simulink model "example_frictions"  (R2023b)
settings: Solver=FixedStepAuto  StartTime=0.0  StopTime=10.0  FixedStep=1/100  RelTol=1e-3
settings Model: Creator=Moi  LastModifiedBy=T0144666
settings OptimizationCC: ReuseModelBlockBuffer=off

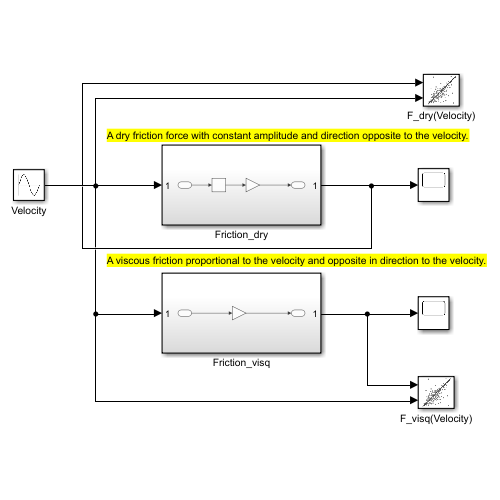
[thumbnail: Simulink's stored preview of the top-level diagram]
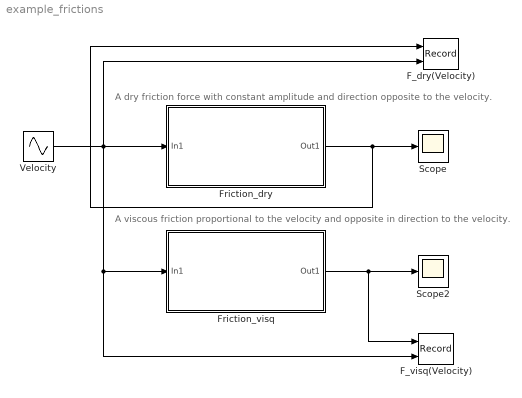
== system example_frictions ==
  note: A dry friction force with constant amplitude and direction opposite to the velocity.
  note: A viscous friction proportional to the velocity and opposite in direction to the velocity.
  F_dry(Velocity) : Record  FileSettingsInternal="{\"entries\":[{\"content\":{\"excelSettings\":{\"content\":{},\"type\":\"Streamout.ExcelSettings\"}},\"type\":\"Streamout.FileSettingStorage\",\"uuid\":\"\"}],\"packageUris\":[\"http:\\/\\/schema.mathworks.com\\/mf0\\/streamout_blocks\\/R2020a\"],\"version\":\"1.0\"}"  Layout=[1 1]  SignalsInternal="{\"entries\":[{\"content\":{\"signals\":[{\"content\":{\"blockPath\":[],\"dimensions\":[1],\"domain\":\"\",\"lineColor\":\"#a2142f\",\"plots\":[1],\"port\":1,\"signalID\":16,\"signalName\":\"frottement_sec\"},\"type\":\"RecordBlkView.Signal\",\"uuid\":\"\"},{\"content\":{\"blockPath\":[],\"dimensions\":[1],\"domain\":\"\",\"lineColor\":\"#139fff\",\"plots\":[1],\"port\":2,\"signalID\":19,\"signalName\":\"vitesse\"},\"type\":\"RecordBlkView.Signal\",\"uuid\":\"\"}]},\"type\":\"RecordBlkView.InputSignals\",\"uuid\":\"\"}],\"packageUris\":[\"http:\\/\\/schema.mathworks.com\\/mf0\\/streamout_blocks\\/R2020a\"],\"version\":\"1.0\"}"  VisualizationBindings="{\"xyplotplugin\":{\"info\":[{\"series\":[{\"bindingParametersList\":[{\"parameter\":\"X-Axis\",\"signalID\":19,\"signalName\":\"vitesse\"},{\"parameter\":\"Y-Axis\",\"signalID\":16,\"signalName\":\"frottement_sec\"}],\"seriesID\":52232}],\"subplotID\":1}]}}"  CompatibilityTag=XY
  F_visq(Velocity) : Record  FileSettingsInternal="{\"entries\":[{\"content\":{\"excelSettings\":{\"content\":{},\"type\":\"Streamout.ExcelSettings\"}},\"type\":\"Streamout.FileSettingStorage\",\"uuid\":\"\"}],\"packageUris\":[\"http:\\/\\/schema.mathworks.com\\/mf0\\/streamout_blocks\\/R2020a\"],\"version\":\"1.0\"}"  Layout=[1 1]  SignalsInternal="{\"entries\":[{\"content\":{\"signals\":[{\"content\":{\"blockPath\":[],\"dimensions\":[1],\"domain\":\"\",\"lineColor\":\"#ff6929\",\"plots\":[1],\"port\":1,\"signalID\":8,\"signalName\":\"frottement_visqueux\"},\"type\":\"RecordBlkView.Signal\",\"uuid\":\"\"},{\"content\":{\"blockPath\":[],\"dimensions\":[1],\"domain\":\"\",\"lineColor\":\"#b746ff\",\"plots\":[1],\"port\":2,\"signalID\":11,\"signalName\":\"vitesse\"},\"type\":\"RecordBlkView.Signal\",\"uuid\":\"\"}]},\"type\":\"RecordBlkView.InputSignals\",\"uuid\":\"\"}],\"packageUris\":[\"http:\\/\\/schema.mathworks.com\\/mf0\\/streamout_blocks\\/R2020a\"],\"version\":\"1.0\"}"  VisualizationBindings="{\"xyplotplugin\":{\"info\":[{\"series\":[{\"bindingParametersList\":[{\"parameter\":\"X-Axis\",\"signalID\":11,\"signalName\":\"vitesse\"},{\"parameter\":\"Y-Axis\",\"signalID\":8,\"signalName\":\"frottement_visqueux\"}],\"seriesID\":60797}],\"subplotID\":1}]}}"  CompatibilityTag=XY
  Friction_dry : Subsystem
  Friction_visq : Subsystem
  Scope : Scope
  Scope2 : Scope
  Velocity : Sin  Amplitude=3  SampleTime=0
  wires:
  Velocity/1 -> F_visq(Velocity)/2, Friction_visq/1(In1), Friction_dry/1(In1), F_dry(Velocity)/2
  Friction_dry/1(Out1) -> F_dry(Velocity)/1, Scope/1
  Friction_visq/1(Out1) -> F_visq(Velocity)/1, Scope2/1

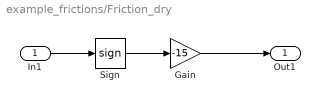
== system example_frictions/Friction_dry ==
  In1 : Inport
  Gain : Gain  Gain=-15
  Sign : Signum
  Out1 : Outport
  wires:
  Sign/1 -> Gain/1
  In1/1 -> Sign/1
  Gain/1 -> Out1/1

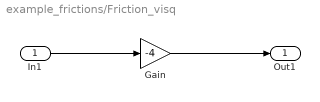
== system example_frictions/Friction_visq ==
  In1 : Inport
  Gain : Gain  Gain=-4
  Out1 : Outport
  wires:
  Gain/1 -> Out1/1
  In1/1 -> Gain/1
